simulink library "sm_wheel_loader_lib"  (R2025a)
settings: Solver=VariableStepAuto  StartTime=0.0  StopTime=10.0  RelTol=1e-3
undefined symbols (not defined in the file): AToTOrificeVector, BiPOrificeVector, boomHEArea, boomREArea, BToTOrificeVector, fluids, GRake, GToothL, GToothR, HMPST, HydFcnParams, logLoad, Position, PToAOrificeVector, PToBOrificeVector, RakeL, RakeR, testInput, Wheel_Loader, X, Y, Z
libraries: sm_lib x694, fl_lib x183, nesl_utility x74, SimscapeFluids_lib x62, sdl_lib x25, cvt_components_lib x25, simulink_extras x5, $bdroot x4, wheel_loader_contact_lib x4, ee_lib x2, SignalEditorBlockLib x1, batteryecm_lib x1
(part 17 of 26)

== system sm_wheel_loader_lib/Wheel Loader Vehicle/Driveline/Driveline/Driveline 3D/Planetary FL ==
  Carrier : Subsystem  Tag=E5EDD8BF-BFC4-A349-9C21-406C76E99105
      mask Display: image('sm_wheel_loader_wheelhub_carrier_IMAGE.png')
  Constraint Ring P1 : sm_lib/Gears and Couplings/Gears/Common Gear Constraint  GearType=Internal  SpecificationType=CenterDistanceRatio  CenterDistance=0.0378618750  CenterDistanceUnits=m  GearRatio=87/30  BaseGearRadius=10.0  BaseGearRadiusUnits=cm  FollGearRadius=10.0  FollGearRadiusUnits=cm
  Constraint Ring P2 : sm_lib/Gears and Couplings/Gears/Common Gear Constraint  GearType=Internal  SpecificationType=CenterDistanceRatio  CenterDistance=0.0378618750  CenterDistanceUnits=m  GearRatio=87/30  BaseGearRadius=10.0  BaseGearRadiusUnits=cm  FollGearRadius=10.0  FollGearRadiusUnits=cm
  "Constraint Ring P3 " : sm_lib/Gears and Couplings/Gears/Common Gear Constraint  GearType=Internal  SpecificationType=CenterDistanceRatio  CenterDistance=0.0378618750  CenterDistanceUnits=m  GearRatio=87/30  BaseGearRadius=10.0  BaseGearRadiusUnits=cm  FollGearRadius=10.0  FollGearRadiusUnits=cm
  Constraint Sun P1 : sm_lib/Gears and Couplings/Gears/Common Gear Constraint  GearType=External  SpecificationType=CenterDistanceRatio  CenterDistance=0.0378618750  CenterDistanceUnits=m  GearRatio=30/24  BaseGearRadius=10.0  BaseGearRadiusUnits=cm  FollGearRadius=10.0  FollGearRadiusUnits=cm
  Constraint Sun P2 : sm_lib/Gears and Couplings/Gears/Common Gear Constraint  GearType=External  SpecificationType=CenterDistanceRatio  CenterDistance=0.0378618750  CenterDistanceUnits=m  GearRatio=30/24  BaseGearRadius=10.0  BaseGearRadiusUnits=cm  FollGearRadius=10.0  FollGearRadiusUnits=cm
  Constraint Sun P3 : sm_lib/Gears and Couplings/Gears/Common Gear Constraint  GearType=External  SpecificationType=CenterDistanceRatio  CenterDistance=0.0378618750  CenterDistanceUnits=m  GearRatio=30/24  BaseGearRadius=10.0  BaseGearRadiusUnits=cm  FollGearRadius=10.0  FollGearRadiusUnits=cm
  Planet 1 : Subsystem  Tag=FDEB1220-0511-4448-BDCD-A712481434B5
      settings: PortSchema="{\"entries\":[{\"content\":{\"sides\":[{\"content\":{\"connectorIds\":[\"LConn1\"]},\"type\":\"ConnectorPlacement.EquallySpacedRectSide\",\"uuid\":\"a60cb0c8-d211-4b25-8f67-7c487f4c42c9\"},{\"content\":{\"connectorIds\":[\"RConn1\"],\"side\":\"RIGHT\"},\"type\":\"ConnectorPlacement.EquallySpacedRectSide\",\"uuid\":\"60889ee7-a0f0-4123-a185-e299563c3562\"},{\"content\":{\"side\":\"TOP\"},\"type\":\"ConnectorPlacement.EquallySpacedRectSide\",\"uuid\":\"edc0ab5f-d81e-451a-97cb-6ac30fa26360\"},{\"content\":{\"connectorIds\":[\"RConn2\"],\"side\":\"BOTTOM\"},\"type\":\"ConnectorPlacement.EquallySpacedRectSide\",\"uuid\":\"6e0ec680-9dd2-41d4-9c2f-6fb875b64084\"}]},\"type\":\"ConnectorPlacement.EquallySpacedConnector\",\"uuid\":\"30ed9e8a-6d07-4a78-9a09-a3c08f1b9746\"}],\"packageUris\":[\"http://schema.mathworks.com/mf0/Connector/R2020b\"],\"version\":\"1.0\"}"
      mask Display: image('sm_wheel_loader_wheelhub_planet1_IMAGE.png')
  Planet 2 : Subsystem  Tag=FDEB1220-0511-4448-BDCD-A712481434B5
      settings: PortSchema="{\"entries\":[{\"content\":{\"sides\":[{\"content\":{\"connectorIds\":[\"LConn1\"]},\"type\":\"ConnectorPlacement.EquallySpacedRectSide\",\"uuid\":\"a60cb0c8-d211-4b25-8f67-7c487f4c42c9\"},{\"content\":{\"connectorIds\":[\"RConn1\"],\"side\":\"RIGHT\"},\"type\":\"ConnectorPlacement.EquallySpacedRectSide\",\"uuid\":\"60889ee7-a0f0-4123-a185-e299563c3562\"},{\"content\":{\"side\":\"TOP\"},\"type\":\"ConnectorPlacement.EquallySpacedRectSide\",\"uuid\":\"edc0ab5f-d81e-451a-97cb-6ac30fa26360\"},{\"content\":{\"connectorIds\":[\"RConn2\"],\"side\":\"BOTTOM\"},\"type\":\"ConnectorPlacement.EquallySpacedRectSide\",\"uuid\":\"6585e4ce-f4ae-4617-9d75-f4dabf4bb1a9\"}]},\"type\":\"ConnectorPlacement.EquallySpacedConnector\",\"uuid\":\"30ed9e8a-6d07-4a78-9a09-a3c08f1b9746\"}],\"packageUris\":[\"http://schema.mathworks.com/mf0/Connector/R2020b\"],\"version\":\"1.0\"}"
      mask Display: image('sm_wheel_loader_wheelhub_planet2_IMAGE.png')
  Planet 3 : Subsystem  Tag=FDEB1220-0511-4448-BDCD-A712481434B5
      settings: PortSchema="{\"entries\":[{\"content\":{\"sides\":[{\"content\":{\"connectorIds\":[\"LConn1\"]},\"type\":\"ConnectorPlacement.EquallySpacedRectSide\",\"uuid\":\"a60cb0c8-d211-4b25-8f67-7c487f4c42c9\"},{\"content\":{\"connectorIds\":[\"RConn1\"],\"side\":\"RIGHT\"},\"type\":\"ConnectorPlacement.EquallySpacedRectSide\",\"uuid\":\"60889ee7-a0f0-4123-a185-e299563c3562\"},{\"content\":{\"side\":\"TOP\"},\"type\":\"ConnectorPlacement.EquallySpacedRectSide\",\"uuid\":\"edc0ab5f-d81e-451a-97cb-6ac30fa26360\"},{\"content\":{\"connectorIds\":[\"RConn2\"],\"side\":\"BOTTOM\"},\"type\":\"ConnectorPlacement.EquallySpacedRectSide\",\"uuid\":\"99038176-9f1e-46e5-b67f-0969ce6d6412\"}]},\"type\":\"ConnectorPlacement.EquallySpacedConnector\",\"uuid\":\"30ed9e8a-6d07-4a78-9a09-a3c08f1b9746\"}],\"packageUris\":[\"http://schema.mathworks.com/mf0/Connector/R2020b\"],\"version\":\"1.0\"}"
      mask Display: image('sm_wheel_loader_wheelhub_planet3_IMAGE.png')
  Revolute Carrier P1 : sm_lib/Joints/Revolute Joint  JointMode=Normal  CompositeWrenchDir=FollowerOnBase  CompositeWrenchFrame=BaseFrame  SenseConstraintForce=off  SenseConstraintTorque=off  SenseTotalForce=off  SenseTotalTorque=off  PositionTargetSpecify=off  PositionTargetPriority=High  PositionTargetValue=0  PositionTargetValueUnits=deg  VelocityTargetSpecify=off  VelocityTargetPriority=High  VelocityTargetValue=0  VelocityTargetValueUnits=deg/s  EquilibriumPosition=0  EquilibriumPositionUnits=deg  SpringStiffness=0  SpringStiffnessUnits=N*m/deg  DampingCoefficient=0  DampingCoefficientUnits=N*m/(deg/s)  LowerLimitSpecify=off  LowerLimitBound=-90  LowerLimitBoundUnits=deg  LowerLimitStiffness=1e4  LowerLimitStiffnessUnits=N*m/deg  LowerLimitDamping=10  LowerLimitDampingUnits=N*m/(deg/s)  LowerLimitTransitionRegionWidth=0.1  LowerLimitTransitionRegionWidthUnits=deg  UpperLimitSpecify=off  UpperLimitBound=90  UpperLimitBoundUnits=deg  UpperLimitStiffness=1e4  UpperLimitStiffnessUnits=N*m/deg  UpperLimitDamping=10  UpperLimitDampingUnits=N*m/(deg/s)  UpperLimitTransitionRegionWidth=0.1  UpperLimitTransitionRegionWidthUnits=deg  TorqueActuationMode=NoTorque  MotionActuationMode=ComputedMotion  SensePosition=off  SenseVelocity=off  SenseAcceleration=off  SenseTorqueForce=off  SenseLowerLimitTorqueForce=off  SenseUpperLimitTorqueForce=off
  Revolute Carrier P2 : sm_lib/Joints/Revolute Joint  JointMode=Normal  CompositeWrenchDir=FollowerOnBase  CompositeWrenchFrame=BaseFrame  SenseConstraintForce=off  SenseConstraintTorque=off  SenseTotalForce=off  SenseTotalTorque=off  PositionTargetSpecify=off  PositionTargetPriority=High  PositionTargetValue=0  PositionTargetValueUnits=deg  VelocityTargetSpecify=off  VelocityTargetPriority=High  VelocityTargetValue=0  VelocityTargetValueUnits=deg/s  EquilibriumPosition=0  EquilibriumPositionUnits=deg  SpringStiffness=0  SpringStiffnessUnits=N*m/deg  DampingCoefficient=0  DampingCoefficientUnits=N*m/(deg/s)  LowerLimitSpecify=off  LowerLimitBound=-90  LowerLimitBoundUnits=deg  LowerLimitStiffness=1e4  LowerLimitStiffnessUnits=N*m/deg  LowerLimitDamping=10  LowerLimitDampingUnits=N*m/(deg/s)  LowerLimitTransitionRegionWidth=0.1  LowerLimitTransitionRegionWidthUnits=deg  UpperLimitSpecify=off  UpperLimitBound=90  UpperLimitBoundUnits=deg  UpperLimitStiffness=1e4  UpperLimitStiffnessUnits=N*m/deg  UpperLimitDamping=10  UpperLimitDampingUnits=N*m/(deg/s)  UpperLimitTransitionRegionWidth=0.1  UpperLimitTransitionRegionWidthUnits=deg  TorqueActuationMode=NoTorque  MotionActuationMode=ComputedMotion  SensePosition=off  SenseVelocity=off  SenseAcceleration=off  SenseTorqueForce=off  SenseLowerLimitTorqueForce=off  SenseUpperLimitTorqueForce=off
  Revolute Carrier P3 : sm_lib/Joints/Revolute Joint  JointMode=Normal  CompositeWrenchDir=FollowerOnBase  CompositeWrenchFrame=BaseFrame  SenseConstraintForce=off  SenseConstraintTorque=off  SenseTotalForce=off  SenseTotalTorque=off  PositionTargetSpecify=off  PositionTargetPriority=High  PositionTargetValue=0  PositionTargetValueUnits=deg  VelocityTargetSpecify=off  VelocityTargetPriority=High  VelocityTargetValue=0  VelocityTargetValueUnits=deg/s  EquilibriumPosition=0  EquilibriumPositionUnits=deg  SpringStiffness=0  SpringStiffnessUnits=N*m/deg  DampingCoefficient=0  DampingCoefficientUnits=N*m/(deg/s)  LowerLimitSpecify=off  LowerLimitBound=-90  LowerLimitBoundUnits=deg  LowerLimitStiffness=1e4  LowerLimitStiffnessUnits=N*m/deg  LowerLimitDamping=10  LowerLimitDampingUnits=N*m/(deg/s)  LowerLimitTransitionRegionWidth=0.1  LowerLimitTransitionRegionWidthUnits=deg  UpperLimitSpecify=off  UpperLimitBound=90  UpperLimitBoundUnits=deg  UpperLimitStiffness=1e4  UpperLimitStiffnessUnits=N*m/deg  UpperLimitDamping=10  UpperLimitDampingUnits=N*m/(deg/s)  UpperLimitTransitionRegionWidth=0.1  UpperLimitTransitionRegionWidthUnits=deg  TorqueActuationMode=NoTorque  MotionActuationMode=ComputedMotion  SensePosition=off  SenseVelocity=off  SenseAcceleration=off  SenseTorqueForce=off  SenseLowerLimitTorqueForce=off  SenseUpperLimitTorqueForce=off
  Revolute Ring Carrier : sm_lib/Joints/Revolute Joint  JointMode=Normal  CompositeWrenchDir=FollowerOnBase  CompositeWrenchFrame=BaseFrame  SenseConstraintForce=off  SenseConstraintTorque=off  SenseTotalForce=off  SenseTotalTorque=off  PositionTargetSpecify=off  PositionTargetPriority=High  PositionTargetValue=0  PositionTargetValueUnits=deg  VelocityTargetSpecify=off  VelocityTargetPriority=High  VelocityTargetValue=0  VelocityTargetValueUnits=deg/s  EquilibriumPosition=0  EquilibriumPositionUnits=deg  SpringStiffness=0  SpringStiffnessUnits=N*m/deg  DampingCoefficient=0  DampingCoefficientUnits=N*m/(deg/s)  LowerLimitSpecify=off  LowerLimitBound=-90  LowerLimitBoundUnits=deg  LowerLimitStiffness=1e4  LowerLimitStiffnessUnits=N*m/deg  LowerLimitDamping=10  LowerLimitDampingUnits=N*m/(deg/s)  LowerLimitTransitionRegionWidth=0.1  LowerLimitTransitionRegionWidthUnits=deg  UpperLimitSpecify=off  UpperLimitBound=90  UpperLimitBoundUnits=deg  UpperLimitStiffness=1e4  UpperLimitStiffnessUnits=N*m/deg  UpperLimitDamping=10  UpperLimitDampingUnits=N*m/(deg/s)  UpperLimitTransitionRegionWidth=0.1  UpperLimitTransitionRegionWidthUnits=deg  TorqueActuationMode=NoTorque  MotionActuationMode=ComputedMotion  SensePosition=off  SenseVelocity=off  SenseAcceleration=off  SenseTorqueForce=off  SenseLowerLimitTorqueForce=off  SenseUpperLimitTorqueForce=off
  Revolute Ring Sun : sm_lib/Joints/Revolute Joint  JointMode=Normal  CompositeWrenchDir=FollowerOnBase  CompositeWrenchFrame=BaseFrame  SenseConstraintForce=off  SenseConstraintTorque=off  SenseTotalForce=off  SenseTotalTorque=off  PositionTargetSpecify=off  PositionTargetPriority=High  PositionTargetValue=0  PositionTargetValueUnits=deg  VelocityTargetSpecify=off  VelocityTargetPriority=High  VelocityTargetValue=0  VelocityTargetValueUnits=deg/s  EquilibriumPosition=0  EquilibriumPositionUnits=deg  SpringStiffness=0  SpringStiffnessUnits=N*m/deg  DampingCoefficient=0  DampingCoefficientUnits=N*m/(deg/s)  LowerLimitSpecify=off  LowerLimitBound=-90  LowerLimitBoundUnits=deg  LowerLimitStiffness=1e4  LowerLimitStiffnessUnits=N*m/deg  LowerLimitDamping=10  LowerLimitDampingUnits=N*m/(deg/s)  LowerLimitTransitionRegionWidth=0.1  LowerLimitTransitionRegionWidthUnits=deg  UpperLimitSpecify=off  UpperLimitBound=90  UpperLimitBoundUnits=deg  UpperLimitStiffness=1e4  UpperLimitStiffnessUnits=N*m/deg  UpperLimitDamping=10  UpperLimitDampingUnits=N*m/(deg/s)  UpperLimitTransitionRegionWidth=0.1  UpperLimitTransitionRegionWidthUnits=deg  TorqueActuationMode=NoTorque  MotionActuationMode=ComputedMotion  SensePosition=off  SenseVelocity=off  SenseAcceleration=off  SenseTorqueForce=off  SenseLowerLimitTorqueForce=off  SenseUpperLimitTorqueForce=off
  Ring Gear : Subsystem  Tag=B2A6520B-B79A-3144-97C4-6FFE059DED13
      mask Display: image('sm_wheel_loader_wheelhub_ring_IMAGE.png')
  Sun Gear : Subsystem  Tag=8B7F22EE-9A8C-C248-9BA7-4E4096F4C17B
      mask Display: image('sm_wheel_loader_wheelhub_sun_IMAGE.png')
  "S  " : PMIOPort  Side=Right
  S1 : PMIOPort  Port=2  Side=Left
  C1 : PMIOPort  Port=3  Side=Left
  "C  " : PMIOPort  Port=4  Side=Right
  "R  " : PMIOPort  Port=5  Side=Right
  R1 : PMIOPort  Port=6  Side=Left
  connections:
  S1/RConn1 -- Sun Gear/LConn1 -- "S  "/RConn1
  Carrier/RConn1 -- Revolute Ring Carrier/RConn1 -- "C  "/RConn1 -- C1/RConn1
  Planet 3/RConn2 -- Revolute Carrier P3/RConn1
  Planet 3/RConn1 -- "Constraint Ring P3 "/LConn1
  Planet 3/LConn1 -- Constraint Sun P3/RConn1
  Planet 2/RConn2 -- Revolute Carrier P2/RConn1
  Planet 2/RConn1 -- Constraint Ring P2/LConn1
  Planet 2/LConn1 -- Constraint Sun P2/RConn1
  Constraint Sun P1/RConn1 -- Planet 1/LConn1
  Revolute Carrier P1/RConn1 -- Planet 1/RConn2
  Carrier/LConn3 -- Revolute Carrier P3/LConn1
  Carrier/LConn2 -- Revolute Carrier P2/LConn1
  Carrier/LConn1 -- Revolute Carrier P1/LConn1
  Revolute Ring Carrier/LConn1 -- "R  "/RConn1 -- R1/RConn1 -- Ring Gear/LConn1 -- Revolute Ring Sun/LConn1 -- Constraint Ring P1/RConn1 -- "Constraint Ring P3 "/RConn1 -- Constraint Ring P2/RConn1
  Planet 1/RConn1 -- Constraint Ring P1/LConn1
  Constraint Sun P3/LConn1 -- Constraint Sun P2/LConn1 -- Constraint Sun P1/LConn1 -- Sun Gear/RConn1 -- Revolute Ring Sun/RConn1

== system sm_wheel_loader_lib/Wheel Loader Vehicle/Driveline/Driveline/Driveline 3D/Planetary FR ==
  Carrier : Subsystem  Tag=E5EDD8BF-BFC4-A349-9C21-406C76E99105
      mask Display: image('sm_wheel_loader_wheelhub_carrier_IMAGE.png')
  Constraint Ring P1 : sm_lib/Gears and Couplings/Gears/Common Gear Constraint  GearType=Internal  SpecificationType=CenterDistanceRatio  CenterDistance=0.0378618750  CenterDistanceUnits=m  GearRatio=87/30  BaseGearRadius=10.0  BaseGearRadiusUnits=cm  FollGearRadius=10.0  FollGearRadiusUnits=cm
  Constraint Ring P2 : sm_lib/Gears and Couplings/Gears/Common Gear Constraint  GearType=Internal  SpecificationType=CenterDistanceRatio  CenterDistance=0.0378618750  CenterDistanceUnits=m  GearRatio=87/30  BaseGearRadius=10.0  BaseGearRadiusUnits=cm  FollGearRadius=10.0  FollGearRadiusUnits=cm
  "Constraint Ring P3 " : sm_lib/Gears and Couplings/Gears/Common Gear Constraint  GearType=Internal  SpecificationType=CenterDistanceRatio  CenterDistance=0.0378618750  CenterDistanceUnits=m  GearRatio=87/30  BaseGearRadius=10.0  BaseGearRadiusUnits=cm  FollGearRadius=10.0  FollGearRadiusUnits=cm
  Constraint Sun P1 : sm_lib/Gears and Couplings/Gears/Common Gear Constraint  GearType=External  SpecificationType=CenterDistanceRatio  CenterDistance=0.0378618750  CenterDistanceUnits=m  GearRatio=30/24  BaseGearRadius=10.0  BaseGearRadiusUnits=cm  FollGearRadius=10.0  FollGearRadiusUnits=cm
  Constraint Sun P2 : sm_lib/Gears and Couplings/Gears/Common Gear Constraint  GearType=External  SpecificationType=CenterDistanceRatio  CenterDistance=0.0378618750  CenterDistanceUnits=m  GearRatio=30/24  BaseGearRadius=10.0  BaseGearRadiusUnits=cm  FollGearRadius=10.0  FollGearRadiusUnits=cm
  Constraint Sun P3 : sm_lib/Gears and Couplings/Gears/Common Gear Constraint  GearType=External  SpecificationType=CenterDistanceRatio  CenterDistance=0.0378618750  CenterDistanceUnits=m  GearRatio=30/24  BaseGearRadius=10.0  BaseGearRadiusUnits=cm  FollGearRadius=10.0  FollGearRadiusUnits=cm
  Planet 1 : Subsystem  Tag=FDEB1220-0511-4448-BDCD-A712481434B5
      settings: PortSchema="{\"entries\":[{\"content\":{\"sides\":[{\"content\":{\"connectorIds\":[\"LConn1\"]},\"type\":\"ConnectorPlacement.EquallySpacedRectSide\",\"uuid\":\"a60cb0c8-d211-4b25-8f67-7c487f4c42c9\"},{\"content\":{\"connectorIds\":[\"RConn1\"],\"side\":\"RIGHT\"},\"type\":\"ConnectorPlacement.EquallySpacedRectSide\",\"uuid\":\"60889ee7-a0f0-4123-a185-e299563c3562\"},{\"content\":{\"side\":\"TOP\"},\"type\":\"ConnectorPlacement.EquallySpacedRectSide\",\"uuid\":\"edc0ab5f-d81e-451a-97cb-6ac30fa26360\"},{\"content\":{\"connectorIds\":[\"RConn2\"],\"side\":\"BOTTOM\"},\"type\":\"ConnectorPlacement.EquallySpacedRectSide\",\"uuid\":\"6e0ec680-9dd2-41d4-9c2f-6fb875b64084\"}]},\"type\":\"ConnectorPlacement.EquallySpacedConnector\",\"uuid\":\"30ed9e8a-6d07-4a78-9a09-a3c08f1b9746\"}],\"packageUris\":[\"http://schema.mathworks.com/mf0/Connector/R2020b\"],\"version\":\"1.0\"}"
      mask Display: image('sm_wheel_loader_wheelhub_planet1_IMAGE.png')
  Planet 2 : Subsystem  Tag=FDEB1220-0511-4448-BDCD-A712481434B5
      settings: PortSchema="{\"entries\":[{\"content\":{\"sides\":[{\"content\":{\"connectorIds\":[\"LConn1\"]},\"type\":\"ConnectorPlacement.EquallySpacedRectSide\",\"uuid\":\"a60cb0c8-d211-4b25-8f67-7c487f4c42c9\"},{\"content\":{\"connectorIds\":[\"RConn1\"],\"side\":\"RIGHT\"},\"type\":\"ConnectorPlacement.EquallySpacedRectSide\",\"uuid\":\"60889ee7-a0f0-4123-a185-e299563c3562\"},{\"content\":{\"side\":\"TOP\"},\"type\":\"ConnectorPlacement.EquallySpacedRectSide\",\"uuid\":\"edc0ab5f-d81e-451a-97cb-6ac30fa26360\"},{\"content\":{\"connectorIds\":[\"RConn2\"],\"side\":\"BOTTOM\"},\"type\":\"ConnectorPlacement.EquallySpacedRectSide\",\"uuid\":\"6585e4ce-f4ae-4617-9d75-f4dabf4bb1a9\"}]},\"type\":\"ConnectorPlacement.EquallySpacedConnector\",\"uuid\":\"30ed9e8a-6d07-4a78-9a09-a3c08f1b9746\"}],\"packageUris\":[\"http://schema.mathworks.com/mf0/Connector/R2020b\"],\"version\":\"1.0\"}"
      mask Display: image('sm_wheel_loader_wheelhub_planet2_IMAGE.png')
  Planet 3 : Subsystem  Tag=FDEB1220-0511-4448-BDCD-A712481434B5
      settings: PortSchema="{\"entries\":[{\"content\":{\"sides\":[{\"content\":{\"connectorIds\":[\"LConn1\"]},\"type\":\"ConnectorPlacement.EquallySpacedRectSide\",\"uuid\":\"a60cb0c8-d211-4b25-8f67-7c487f4c42c9\"},{\"content\":{\"connectorIds\":[\"RConn1\"],\"side\":\"RIGHT\"},\"type\":\"ConnectorPlacement.EquallySpacedRectSide\",\"uuid\":\"60889ee7-a0f0-4123-a185-e299563c3562\"},{\"content\":{\"side\":\"TOP\"},\"type\":\"ConnectorPlacement.EquallySpacedRectSide\",\"uuid\":\"edc0ab5f-d81e-451a-97cb-6ac30fa26360\"},{\"content\":{\"connectorIds\":[\"RConn2\"],\"side\":\"BOTTOM\"},\"type\":\"ConnectorPlacement.EquallySpacedRectSide\",\"uuid\":\"99038176-9f1e-46e5-b67f-0969ce6d6412\"}]},\"type\":\"ConnectorPlacement.EquallySpacedConnector\",\"uuid\":\"30ed9e8a-6d07-4a78-9a09-a3c08f1b9746\"}],\"packageUris\":[\"http://schema.mathworks.com/mf0/Connector/R2020b\"],\"version\":\"1.0\"}"
      mask Display: image('sm_wheel_loader_wheelhub_planet3_IMAGE.png')
  Revolute Carrier P1 : sm_lib/Joints/Revolute Joint  JointMode=Normal  CompositeWrenchDir=FollowerOnBase  CompositeWrenchFrame=BaseFrame  SenseConstraintForce=off  SenseConstraintTorque=off  SenseTotalForce=off  SenseTotalTorque=off  PositionTargetSpecify=off  PositionTargetPriority=High  PositionTargetValue=0  PositionTargetValueUnits=deg  VelocityTargetSpecify=off  VelocityTargetPriority=High  VelocityTargetValue=0  VelocityTargetValueUnits=deg/s  EquilibriumPosition=0  EquilibriumPositionUnits=deg  SpringStiffness=0  SpringStiffnessUnits=N*m/deg  DampingCoefficient=0  DampingCoefficientUnits=N*m/(deg/s)  LowerLimitSpecify=off  LowerLimitBound=-90  LowerLimitBoundUnits=deg  LowerLimitStiffness=1e4  LowerLimitStiffnessUnits=N*m/deg  LowerLimitDamping=10  LowerLimitDampingUnits=N*m/(deg/s)  LowerLimitTransitionRegionWidth=0.1  LowerLimitTransitionRegionWidthUnits=deg  UpperLimitSpecify=off  UpperLimitBound=90  UpperLimitBoundUnits=deg  UpperLimitStiffness=1e4  UpperLimitStiffnessUnits=N*m/deg  UpperLimitDamping=10  UpperLimitDampingUnits=N*m/(deg/s)  UpperLimitTransitionRegionWidth=0.1  UpperLimitTransitionRegionWidthUnits=deg  TorqueActuationMode=NoTorque  MotionActuationMode=ComputedMotion  SensePosition=off  SenseVelocity=off  SenseAcceleration=off  SenseTorqueForce=off  SenseLowerLimitTorqueForce=off  SenseUpperLimitTorqueForce=off
  Revolute Carrier P2 : sm_lib/Joints/Revolute Joint  JointMode=Normal  CompositeWrenchDir=FollowerOnBase  CompositeWrenchFrame=BaseFrame  SenseConstraintForce=off  SenseConstraintTorque=off  SenseTotalForce=off  SenseTotalTorque=off  PositionTargetSpecify=off  PositionTargetPriority=High  PositionTargetValue=0  PositionTargetValueUnits=deg  VelocityTargetSpecify=off  VelocityTargetPriority=High  VelocityTargetValue=0  VelocityTargetValueUnits=deg/s  EquilibriumPosition=0  EquilibriumPositionUnits=deg  SpringStiffness=0  SpringStiffnessUnits=N*m/deg  DampingCoefficient=0  DampingCoefficientUnits=N*m/(deg/s)  LowerLimitSpecify=off  LowerLimitBound=-90  LowerLimitBoundUnits=deg  LowerLimitStiffness=1e4  LowerLimitStiffnessUnits=N*m/deg  LowerLimitDamping=10  LowerLimitDampingUnits=N*m/(deg/s)  LowerLimitTransitionRegionWidth=0.1  LowerLimitTransitionRegionWidthUnits=deg  UpperLimitSpecify=off  UpperLimitBound=90  UpperLimitBoundUnits=deg  UpperLimitStiffness=1e4  UpperLimitStiffnessUnits=N*m/deg  UpperLimitDamping=10  UpperLimitDampingUnits=N*m/(deg/s)  UpperLimitTransitionRegionWidth=0.1  UpperLimitTransitionRegionWidthUnits=deg  TorqueActuationMode=NoTorque  MotionActuationMode=ComputedMotion  SensePosition=off  SenseVelocity=off  SenseAcceleration=off  SenseTorqueForce=off  SenseLowerLimitTorqueForce=off  SenseUpperLimitTorqueForce=off
  Revolute Carrier P3 : sm_lib/Joints/Revolute Joint  JointMode=Normal  CompositeWrenchDir=FollowerOnBase  CompositeWrenchFrame=BaseFrame  SenseConstraintForce=off  SenseConstraintTorque=off  SenseTotalForce=off  SenseTotalTorque=off  PositionTargetSpecify=off  PositionTargetPriority=High  PositionTargetValue=0  PositionTargetValueUnits=deg  VelocityTargetSpecify=off  VelocityTargetPriority=High  VelocityTargetValue=0  VelocityTargetValueUnits=deg/s  EquilibriumPosition=0  EquilibriumPositionUnits=deg  SpringStiffness=0  SpringStiffnessUnits=N*m/deg  DampingCoefficient=0  DampingCoefficientUnits=N*m/(deg/s)  LowerLimitSpecify=off  LowerLimitBound=-90  LowerLimitBoundUnits=deg  LowerLimitStiffness=1e4  LowerLimitStiffnessUnits=N*m/deg  LowerLimitDamping=10  LowerLimitDampingUnits=N*m/(deg/s)  LowerLimitTransitionRegionWidth=0.1  LowerLimitTransitionRegionWidthUnits=deg  UpperLimitSpecify=off  UpperLimitBound=90  UpperLimitBoundUnits=deg  UpperLimitStiffness=1e4  UpperLimitStiffnessUnits=N*m/deg  UpperLimitDamping=10  UpperLimitDampingUnits=N*m/(deg/s)  UpperLimitTransitionRegionWidth=0.1  UpperLimitTransitionRegionWidthUnits=deg  TorqueActuationMode=NoTorque  MotionActuationMode=ComputedMotion  SensePosition=off  SenseVelocity=off  SenseAcceleration=off  SenseTorqueForce=off  SenseLowerLimitTorqueForce=off  SenseUpperLimitTorqueForce=off
  Revolute Ring Carrier : sm_lib/Joints/Revolute Joint  JointMode=Normal  CompositeWrenchDir=FollowerOnBase  CompositeWrenchFrame=BaseFrame  SenseConstraintForce=off  SenseConstraintTorque=off  SenseTotalForce=off  SenseTotalTorque=off  PositionTargetSpecify=off  PositionTargetPriority=High  PositionTargetValue=0  PositionTargetValueUnits=deg  VelocityTargetSpecify=off  VelocityTargetPriority=High  VelocityTargetValue=0  VelocityTargetValueUnits=deg/s  EquilibriumPosition=0  EquilibriumPositionUnits=deg  SpringStiffness=0  SpringStiffnessUnits=N*m/deg  DampingCoefficient=0  DampingCoefficientUnits=N*m/(deg/s)  LowerLimitSpecify=off  LowerLimitBound=-90  LowerLimitBoundUnits=deg  LowerLimitStiffness=1e4  LowerLimitStiffnessUnits=N*m/deg  LowerLimitDamping=10  LowerLimitDampingUnits=N*m/(deg/s)  LowerLimitTransitionRegionWidth=0.1  LowerLimitTransitionRegionWidthUnits=deg  UpperLimitSpecify=off  UpperLimitBound=90  UpperLimitBoundUnits=deg  UpperLimitStiffness=1e4  UpperLimitStiffnessUnits=N*m/deg  UpperLimitDamping=10  UpperLimitDampingUnits=N*m/(deg/s)  UpperLimitTransitionRegionWidth=0.1  UpperLimitTransitionRegionWidthUnits=deg  TorqueActuationMode=NoTorque  MotionActuationMode=ComputedMotion  SensePosition=off  SenseVelocity=off  SenseAcceleration=off  SenseTorqueForce=off  SenseLowerLimitTorqueForce=off  SenseUpperLimitTorqueForce=off
  Revolute Ring Sun : sm_lib/Joints/Revolute Joint  JointMode=Normal  CompositeWrenchDir=FollowerOnBase  CompositeWrenchFrame=BaseFrame  SenseConstraintForce=off  SenseConstraintTorque=off  SenseTotalForce=off  SenseTotalTorque=off  PositionTargetSpecify=off  PositionTargetPriority=High  PositionTargetValue=0  PositionTargetValueUnits=deg  VelocityTargetSpecify=off  VelocityTargetPriority=High  VelocityTargetValue=0  VelocityTargetValueUnits=deg/s  EquilibriumPosition=0  EquilibriumPositionUnits=deg  SpringStiffness=0  SpringStiffnessUnits=N*m/deg  DampingCoefficient=0  DampingCoefficientUnits=N*m/(deg/s)  LowerLimitSpecify=off  LowerLimitBound=-90  LowerLimitBoundUnits=deg  LowerLimitStiffness=1e4  LowerLimitStiffnessUnits=N*m/deg  LowerLimitDamping=10  LowerLimitDampingUnits=N*m/(deg/s)  LowerLimitTransitionRegionWidth=0.1  LowerLimitTransitionRegionWidthUnits=deg  UpperLimitSpecify=off  UpperLimitBound=90  UpperLimitBoundUnits=deg  UpperLimitStiffness=1e4  UpperLimitStiffnessUnits=N*m/deg  UpperLimitDamping=10  UpperLimitDampingUnits=N*m/(deg/s)  UpperLimitTransitionRegionWidth=0.1  UpperLimitTransitionRegionWidthUnits=deg  TorqueActuationMode=NoTorque  MotionActuationMode=ComputedMotion  SensePosition=off  SenseVelocity=off  SenseAcceleration=off  SenseTorqueForce=off  SenseLowerLimitTorqueForce=off  SenseUpperLimitTorqueForce=off
  Ring Gear : Subsystem  Tag=B2A6520B-B79A-3144-97C4-6FFE059DED13
      mask Display: image('sm_wheel_loader_wheelhub_ring_IMAGE.png')
  Sun Gear : Subsystem  Tag=8B7F22EE-9A8C-C248-9BA7-4E4096F4C17B
      mask Display: image('sm_wheel_loader_wheelhub_sun_IMAGE.png')
  "S  " : PMIOPort  Side=Right
  S1 : PMIOPort  Port=2  Side=Left
  C1 : PMIOPort  Port=3  Side=Left
  "C  " : PMIOPort  Port=4  Side=Right
  "R  " : PMIOPort  Port=5  Side=Right
  R1 : PMIOPort  Port=6  Side=Left
  connections:
  Constraint Sun P3/LConn1 -- Sun Gear/RConn1 -- Revolute Ring Sun/LConn1 -- Constraint Sun P1/LConn1 -- Constraint Sun P2/LConn1
  Planet 1/RConn1 -- Constraint Ring P1/LConn1
  Constraint Ring P2/RConn1 -- "Constraint Ring P3 "/RConn1 -- Revolute Ring Carrier/RConn1 -- R1/RConn1 -- "R  "/RConn1 -- Ring Gear/LConn1 -- Revolute Ring Sun/RConn1 -- Constraint Ring P1/RConn1
  Carrier/LConn1 -- Revolute Carrier P1/LConn1
  Carrier/LConn2 -- Revolute Carrier P2/LConn1
  Carrier/LConn3 -- Revolute Carrier P3/LConn1
  Revolute Carrier P1/RConn1 -- Planet 1/RConn2
  Constraint Sun P1/RConn1 -- Planet 1/LConn1
  Planet 2/LConn1 -- Constraint Sun P2/RConn1
  Planet 2/RConn1 -- Constraint Ring P2/LConn1
  Planet 2/RConn2 -- Revolute Carrier P2/RConn1
  Planet 3/LConn1 -- Constraint Sun P3/RConn1
  Planet 3/RConn1 -- "Constraint Ring P3 "/LConn1
  Planet 3/RConn2 -- Revolute Carrier P3/RConn1
  Carrier/RConn1 -- C1/RConn1 -- "C  "/RConn1 -- Revolute Ring Carrier/LConn1
  Sun Gear/LConn1 -- S1/RConn1 -- "S  "/RConn1

== system sm_wheel_loader_lib/Wheel Loader Vehicle/Driveline/Driveline/Driveline 3D/Planetary RL ==
  Carrier : Subsystem  Tag=E5EDD8BF-BFC4-A349-9C21-406C76E99105
      mask Display: image('sm_wheel_loader_wheelhub_carrier_IMAGE.png')
  Constraint Ring P1 : sm_lib/Gears and Couplings/Gears/Common Gear Constraint  GearType=Internal  SpecificationType=CenterDistanceRatio  CenterDistance=0.0378618750  CenterDistanceUnits=m  GearRatio=87/30  BaseGearRadius=10.0  BaseGearRadiusUnits=cm  FollGearRadius=10.0  FollGearRadiusUnits=cm
  Constraint Ring P2 : sm_lib/Gears and Couplings/Gears/Common Gear Constraint  GearType=Internal  SpecificationType=CenterDistanceRatio  CenterDistance=0.0378618750  CenterDistanceUnits=m  GearRatio=87/30  BaseGearRadius=10.0  BaseGearRadiusUnits=cm  FollGearRadius=10.0  FollGearRadiusUnits=cm
  "Constraint Ring P3 " : sm_lib/Gears and Couplings/Gears/Common Gear Constraint  GearType=Internal  SpecificationType=CenterDistanceRatio  CenterDistance=0.0378618750  CenterDistanceUnits=m  GearRatio=87/30  BaseGearRadius=10.0  BaseGearRadiusUnits=cm  FollGearRadius=10.0  FollGearRadiusUnits=cm
  Constraint Sun P1 : sm_lib/Gears and Couplings/Gears/Common Gear Constraint  GearType=External  SpecificationType=CenterDistanceRatio  CenterDistance=0.0378618750  CenterDistanceUnits=m  GearRatio=30/24  BaseGearRadius=10.0  BaseGearRadiusUnits=cm  FollGearRadius=10.0  FollGearRadiusUnits=cm
  Constraint Sun P2 : sm_lib/Gears and Couplings/Gears/Common Gear Constraint  GearType=External  SpecificationType=CenterDistanceRatio  CenterDistance=0.0378618750  CenterDistanceUnits=m  GearRatio=30/24  BaseGearRadius=10.0  BaseGearRadiusUnits=cm  FollGearRadius=10.0  FollGearRadiusUnits=cm
  Constraint Sun P3 : sm_lib/Gears and Couplings/Gears/Common Gear Constraint  GearType=External  SpecificationType=CenterDistanceRatio  CenterDistance=0.0378618750  CenterDistanceUnits=m  GearRatio=30/24  BaseGearRadius=10.0  BaseGearRadiusUnits=cm  FollGearRadius=10.0  FollGearRadiusUnits=cm
  Planet 1 : Subsystem  Tag=FDEB1220-0511-4448-BDCD-A712481434B5
      settings: PortSchema="{\"entries\":[{\"content\":{\"sides\":[{\"content\":{\"connectorIds\":[\"LConn1\"]},\"type\":\"ConnectorPlacement.EquallySpacedRectSide\",\"uuid\":\"a60cb0c8-d211-4b25-8f67-7c487f4c42c9\"},{\"content\":{\"connectorIds\":[\"RConn1\"],\"side\":\"RIGHT\"},\"type\":\"ConnectorPlacement.EquallySpacedRectSide\",\"uuid\":\"60889ee7-a0f0-4123-a185-e299563c3562\"},{\"content\":{\"side\":\"TOP\"},\"type\":\"ConnectorPlacement.EquallySpacedRectSide\",\"uuid\":\"edc0ab5f-d81e-451a-97cb-6ac30fa26360\"},{\"content\":{\"connectorIds\":[\"RConn2\"],\"side\":\"BOTTOM\"},\"type\":\"ConnectorPlacement.EquallySpacedRectSide\",\"uuid\":\"6e0ec680-9dd2-41d4-9c2f-6fb875b64084\"}]},\"type\":\"ConnectorPlacement.EquallySpacedConnector\",\"uuid\":\"30ed9e8a-6d07-4a78-9a09-a3c08f1b9746\"}],\"packageUris\":[\"http://schema.mathworks.com/mf0/Connector/R2020b\"],\"version\":\"1.0\"}"
      mask Display: image('sm_wheel_loader_wheelhub_planet1_IMAGE.png')
  Planet 2 : Subsystem  Tag=FDEB1220-0511-4448-BDCD-A712481434B5
      settings: PortSchema="{\"entries\":[{\"content\":{\"sides\":[{\"content\":{\"connectorIds\":[\"LConn1\"]},\"type\":\"ConnectorPlacement.EquallySpacedRectSide\",\"uuid\":\"a60cb0c8-d211-4b25-8f67-7c487f4c42c9\"},{\"content\":{\"connectorIds\":[\"RConn1\"],\"side\":\"RIGHT\"},\"type\":\"ConnectorPlacement.EquallySpacedRectSide\",\"uuid\":\"60889ee7-a0f0-4123-a185-e299563c3562\"},{\"content\":{\"side\":\"TOP\"},\"type\":\"ConnectorPlacement.EquallySpacedRectSide\",\"uuid\":\"edc0ab5f-d81e-451a-97cb-6ac30fa26360\"},{\"content\":{\"connectorIds\":[\"RConn2\"],\"side\":\"BOTTOM\"},\"type\":\"ConnectorPlacement.EquallySpacedRectSide\",\"uuid\":\"6585e4ce-f4ae-4617-9d75-f4dabf4bb1a9\"}]},\"type\":\"ConnectorPlacement.EquallySpacedConnector\",\"uuid\":\"30ed9e8a-6d07-4a78-9a09-a3c08f1b9746\"}],\"packageUris\":[\"http://schema.mathworks.com/mf0/Connector/R2020b\"],\"version\":\"1.0\"}"
      mask Display: image('sm_wheel_loader_wheelhub_planet2_IMAGE.png')
  Planet 3 : Subsystem  Tag=FDEB1220-0511-4448-BDCD-A712481434B5
      settings: PortSchema="{\"entries\":[{\"content\":{\"sides\":[{\"content\":{\"connectorIds\":[\"LConn1\"]},\"type\":\"ConnectorPlacement.EquallySpacedRectSide\",\"uuid\":\"a60cb0c8-d211-4b25-8f67-7c487f4c42c9\"},{\"content\":{\"connectorIds\":[\"RConn1\"],\"side\":\"RIGHT\"},\"type\":\"ConnectorPlacement.EquallySpacedRectSide\",\"uuid\":\"60889ee7-a0f0-4123-a185-e299563c3562\"},{\"content\":{\"side\":\"TOP\"},\"type\":\"ConnectorPlacement.EquallySpacedRectSide\",\"uuid\":\"edc0ab5f-d81e-451a-97cb-6ac30fa26360\"},{\"content\":{\"connectorIds\":[\"RConn2\"],\"side\":\"BOTTOM\"},\"type\":\"ConnectorPlacement.EquallySpacedRectSide\",\"uuid\":\"99038176-9f1e-46e5-b67f-0969ce6d6412\"}]},\"type\":\"ConnectorPlacement.EquallySpacedConnector\",\"uuid\":\"30ed9e8a-6d07-4a78-9a09-a3c08f1b9746\"}],\"packageUris\":[\"http://schema.mathworks.com/mf0/Connector/R2020b\"],\"version\":\"1.0\"}"
      mask Display: image('sm_wheel_loader_wheelhub_planet3_IMAGE.png')
  Revolute Carrier P1 : sm_lib/Joints/Revolute Joint  JointMode=Normal  CompositeWrenchDir=FollowerOnBase  CompositeWrenchFrame=BaseFrame  SenseConstraintForce=off  SenseConstraintTorque=off  SenseTotalForce=off  SenseTotalTorque=off  PositionTargetSpecify=off  PositionTargetPriority=High  PositionTargetValue=0  PositionTargetValueUnits=deg  VelocityTargetSpecify=off  VelocityTargetPriority=High  VelocityTargetValue=0  VelocityTargetValueUnits=deg/s  EquilibriumPosition=0  EquilibriumPositionUnits=deg  SpringStiffness=0  SpringStiffnessUnits=N*m/deg  DampingCoefficient=0  DampingCoefficientUnits=N*m/(deg/s)  LowerLimitSpecify=off  LowerLimitBound=-90  LowerLimitBoundUnits=deg  LowerLimitStiffness=1e4  LowerLimitStiffnessUnits=N*m/deg  LowerLimitDamping=10  LowerLimitDampingUnits=N*m/(deg/s)  LowerLimitTransitionRegionWidth=0.1  LowerLimitTransitionRegionWidthUnits=deg  UpperLimitSpecify=off  UpperLimitBound=90  UpperLimitBoundUnits=deg  UpperLimitStiffness=1e4  UpperLimitStiffnessUnits=N*m/deg  UpperLimitDamping=10  UpperLimitDampingUnits=N*m/(deg/s)  UpperLimitTransitionRegionWidth=0.1  UpperLimitTransitionRegionWidthUnits=deg  TorqueActuationMode=NoTorque  MotionActuationMode=ComputedMotion  SensePosition=off  SenseVelocity=off  SenseAcceleration=off  SenseTorqueForce=off  SenseLowerLimitTorqueForce=off  SenseUpperLimitTorqueForce=off
  Revolute Carrier P2 : sm_lib/Joints/Revolute Joint  JointMode=Normal  CompositeWrenchDir=FollowerOnBase  CompositeWrenchFrame=BaseFrame  SenseConstraintForce=off  SenseConstraintTorque=off  SenseTotalForce=off  SenseTotalTorque=off  PositionTargetSpecify=off  PositionTargetPriority=High  PositionTargetValue=0  PositionTargetValueUnits=deg  VelocityTargetSpecify=off  VelocityTargetPriority=High  VelocityTargetValue=0  VelocityTargetValueUnits=deg/s  EquilibriumPosition=0  EquilibriumPositionUnits=deg  SpringStiffness=0  SpringStiffnessUnits=N*m/deg  DampingCoefficient=0  DampingCoefficientUnits=N*m/(deg/s)  LowerLimitSpecify=off  LowerLimitBound=-90  LowerLimitBoundUnits=deg  LowerLimitStiffness=1e4  LowerLimitStiffnessUnits=N*m/deg  LowerLimitDamping=10  LowerLimitDampingUnits=N*m/(deg/s)  LowerLimitTransitionRegionWidth=0.1  LowerLimitTransitionRegionWidthUnits=deg  UpperLimitSpecify=off  UpperLimitBound=90  UpperLimitBoundUnits=deg  UpperLimitStiffness=1e4  UpperLimitStiffnessUnits=N*m/deg  UpperLimitDamping=10  UpperLimitDampingUnits=N*m/(deg/s)  UpperLimitTransitionRegionWidth=0.1  UpperLimitTransitionRegionWidthUnits=deg  TorqueActuationMode=NoTorque  MotionActuationMode=ComputedMotion  SensePosition=off  SenseVelocity=off  SenseAcceleration=off  SenseTorqueForce=off  SenseLowerLimitTorqueForce=off  SenseUpperLimitTorqueForce=off
  Revolute Carrier P3 : sm_lib/Joints/Revolute Joint  JointMode=Normal  CompositeWrenchDir=FollowerOnBase  CompositeWrenchFrame=BaseFrame  SenseConstraintForce=off  SenseConstraintTorque=off  SenseTotalForce=off  SenseTotalTorque=off  PositionTargetSpecify=off  PositionTargetPriority=High  PositionTargetValue=0  PositionTargetValueUnits=deg  VelocityTargetSpecify=off  VelocityTargetPriority=High  VelocityTargetValue=0  VelocityTargetValueUnits=deg/s  EquilibriumPosition=0  EquilibriumPositionUnits=deg  SpringStiffness=0  SpringStiffnessUnits=N*m/deg  DampingCoefficient=0  DampingCoefficientUnits=N*m/(deg/s)  LowerLimitSpecify=off  LowerLimitBound=-90  LowerLimitBoundUnits=deg  LowerLimitStiffness=1e4  LowerLimitStiffnessUnits=N*m/deg  LowerLimitDamping=10  LowerLimitDampingUnits=N*m/(deg/s)  LowerLimitTransitionRegionWidth=0.1  LowerLimitTransitionRegionWidthUnits=deg  UpperLimitSpecify=off  UpperLimitBound=90  UpperLimitBoundUnits=deg  UpperLimitStiffness=1e4  UpperLimitStiffnessUnits=N*m/deg  UpperLimitDamping=10  UpperLimitDampingUnits=N*m/(deg/s)  UpperLimitTransitionRegionWidth=0.1  UpperLimitTransitionRegionWidthUnits=deg  TorqueActuationMode=NoTorque  MotionActuationMode=ComputedMotion  SensePosition=off  SenseVelocity=off  SenseAcceleration=off  SenseTorqueForce=off  SenseLowerLimitTorqueForce=off  SenseUpperLimitTorqueForce=off
  Revolute Ring Carrier : sm_lib/Joints/Revolute Joint  JointMode=Normal  CompositeWrenchDir=FollowerOnBase  CompositeWrenchFrame=BaseFrame  SenseConstraintForce=off  SenseConstraintTorque=off  SenseTotalForce=off  SenseTotalTorque=off  PositionTargetSpecify=off  PositionTargetPriority=High  PositionTargetValue=0  PositionTargetValueUnits=deg  VelocityTargetSpecify=off  VelocityTargetPriority=High  VelocityTargetValue=0  VelocityTargetValueUnits=deg/s  EquilibriumPosition=0  EquilibriumPositionUnits=deg  SpringStiffness=0  SpringStiffnessUnits=N*m/deg  DampingCoefficient=0  DampingCoefficientUnits=N*m/(deg/s)  LowerLimitSpecify=off  LowerLimitBound=-90  LowerLimitBoundUnits=deg  LowerLimitStiffness=1e4  LowerLimitStiffnessUnits=N*m/deg  LowerLimitDamping=10  LowerLimitDampingUnits=N*m/(deg/s)  LowerLimitTransitionRegionWidth=0.1  LowerLimitTransitionRegionWidthUnits=deg  UpperLimitSpecify=off  UpperLimitBound=90  UpperLimitBoundUnits=deg  UpperLimitStiffness=1e4  UpperLimitStiffnessUnits=N*m/deg  UpperLimitDamping=10  UpperLimitDampingUnits=N*m/(deg/s)  UpperLimitTransitionRegionWidth=0.1  UpperLimitTransitionRegionWidthUnits=deg  TorqueActuationMode=NoTorque  MotionActuationMode=ComputedMotion  SensePosition=off  SenseVelocity=off  SenseAcceleration=off  SenseTorqueForce=off  SenseLowerLimitTorqueForce=off  SenseUpperLimitTorqueForce=off
  Revolute Ring Sun : sm_lib/Joints/Revolute Joint  JointMode=Normal  CompositeWrenchDir=FollowerOnBase  CompositeWrenchFrame=BaseFrame  SenseConstraintForce=off  SenseConstraintTorque=off  SenseTotalForce=off  SenseTotalTorque=off  PositionTargetSpecify=off  PositionTargetPriority=High  PositionTargetValue=0  PositionTargetValueUnits=deg  VelocityTargetSpecify=off  VelocityTargetPriority=High  VelocityTargetValue=0  VelocityTargetValueUnits=deg/s  EquilibriumPosition=0  EquilibriumPositionUnits=deg  SpringStiffness=0  SpringStiffnessUnits=N*m/deg  DampingCoefficient=0  DampingCoefficientUnits=N*m/(deg/s)  LowerLimitSpecify=off  LowerLimitBound=-90  LowerLimitBoundUnits=deg  LowerLimitStiffness=1e4  LowerLimitStiffnessUnits=N*m/deg  LowerLimitDamping=10  LowerLimitDampingUnits=N*m/(deg/s)  LowerLimitTransitionRegionWidth=0.1  LowerLimitTransitionRegionWidthUnits=deg  UpperLimitSpecify=off  UpperLimitBound=90  UpperLimitBoundUnits=deg  UpperLimitStiffness=1e4  UpperLimitStiffnessUnits=N*m/deg  UpperLimitDamping=10  UpperLimitDampingUnits=N*m/(deg/s)  UpperLimitTransitionRegionWidth=0.1  UpperLimitTransitionRegionWidthUnits=deg  TorqueActuationMode=NoTorque  MotionActuationMode=ComputedMotion  SensePosition=off  SenseVelocity=off  SenseAcceleration=off  SenseTorqueForce=off  SenseLowerLimitTorqueForce=off  SenseUpperLimitTorqueForce=off
  Ring Gear : Subsystem  Tag=B2A6520B-B79A-3144-97C4-6FFE059DED13
      mask Display: image('sm_wheel_loader_wheelhub_ring_IMAGE.png')
  Sun Gear : Subsystem  Tag=8B7F22EE-9A8C-C248-9BA7-4E4096F4C17B
      mask Display: image('sm_wheel_loader_wheelhub_sun_IMAGE.png')
  "R  " : PMIOPort  Side=Right
  R1 : PMIOPort  Port=2  Side=Left
  C1 : PMIOPort  Port=3  Side=Left
  "C  " : PMIOPort  Port=4  Side=Right
  "S  " : PMIOPort  Port=5  Side=Right
  S1 : PMIOPort  Port=6  Side=Left
  connections:
  Constraint Sun P3/LConn1 -- Sun Gear/RConn1 -- Revolute Ring Sun/RConn1 -- Constraint Sun P1/LConn1 -- Constraint Sun P2/LConn1
  Planet 1/RConn1 -- Constraint Ring P1/LConn1
  R1/RConn1 -- "R  "/RConn1 -- Revolute Ring Carrier/LConn1 -- Ring Gear/LConn1 -- Revolute Ring Sun/LConn1 -- Constraint Ring P2/RConn1 -- "Constraint Ring P3 "/RConn1 -- Constraint Ring P1/RConn1
  Carrier/RConn1 -- Revolute Carrier P1/LConn1
  Carrier/RConn2 -- Revolute Carrier P2/LConn1
  Carrier/RConn3 -- Revolute Carrier P3/LConn1
  Revolute Carrier P1/RConn1 -- Planet 1/RConn2
  Constraint Sun P1/RConn1 -- Planet 1/LConn1
  Planet 2/LConn1 -- Constraint Sun P2/RConn1
  Planet 2/RConn1 -- Constraint Ring P2/LConn1
  Planet 2/RConn2 -- Revolute Carrier P2/RConn1
  Planet 3/LConn1 -- Constraint Sun P3/RConn1
  Planet 3/RConn1 -- "Constraint Ring P3 "/LConn1
  Planet 3/RConn2 -- Revolute Carrier P3/RConn1
  C1/RConn1 -- "C  "/RConn1 -- Carrier/LConn1 -- Revolute Ring Carrier/RConn1
  Sun Gear/LConn1 -- S1/RConn1 -- "S  "/RConn1
